simulink model "ElectricVehicleThermalManagementWithHeatPump"  (R2024b)
settings: Solver=VariableStepAuto  StartTime=0.0  StopTime=3600  RelTol=1e-3  AbsTol=1e-3
PreLoadFcn:
  | init_nmpc
InitFcn:
  | init_nmpc
model workspace: external: MATLAB File ElectricVehicleThermalManagementWithHeatPumpParameters.m (data not in the file)
values from neighbouring files (symbols this model uses):
  battery_C1_LUT = [1913.6 12447 30609 ... (first row only)    [ElectricVehicleThermalManagementWithHeatPumpParameters.m]
  battery_capacity_LUT = [280.081 276.25 276.392]    [ElectricVehicleThermalManagementWithHeatPumpParameters.m]
  battery_cell_cp = 795    [ElectricVehicleThermalManagementWithHeatPumpParameters.m]
  battery_cell_mass = 2.5    [ElectricVehicleThermalManagementWithHeatPumpParameters.m]
  battery_Em_LUT = [3.4966 3.5057 3.5148 ... (first row only)    [ElectricVehicleThermalManagementWithHeatPumpParameters.m]
  battery_N_cells = 20    [ElectricVehicleThermalManagementWithHeatPumpParameters.m]
  battery_Qe_init = 0    [ElectricVehicleThermalManagementWithHeatPumpParameters.m]
  battery_R0_LUT = [0.0117 0.0085 0.009 ... (first row only)    [ElectricVehicleThermalManagementWithHeatPumpParameters.m]
  battery_R1_LUT = [0.0109 0.0029 0.0013 ... (first row only)    [ElectricVehicleThermalManagementWithHeatPumpParameters.m]
  battery_SOC_LUT = [0; 0.1; 0.25; 0.5; 0.75; 0.9; 1]    [ElectricVehicleThermalManagementWithHeatPumpParameters.m]
  battery_T_init = -10    [ElectricVehicleThermalManagementWithHeatPumpParameters.m]
  battery_temperature_LUT = [5 20 40]    [ElectricVehicleThermalManagementWithHeatPumpParameters.m]
  cabin_duct_area = 0.04    [ElectricVehicleThermalManagementWithHeatPumpParameters.m]
  cabin_T_init = -10    [ElectricVehicleThermalManagementWithHeatPumpParameters.m]
  chiller_area_primary = 0.43982297150257105    (= 0.439822971503)    [ElectricVehicleThermalManagementWithHeatPumpParameters.m]
  chiller_N_baffles = 3    [ElectricVehicleThermalManagementWithHeatPumpParameters.m]
  chiller_N_tubes = 100    [ElectricVehicleThermalManagementWithHeatPumpParameters.m]
  chiller_tube_D = 0.0035    [ElectricVehicleThermalManagementWithHeatPumpParameters.m]
  chiller_tube_L = 0.4    [ElectricVehicleThermalManagementWithHeatPumpParameters.m]
  chiller_wall_conductivity = 240    [ElectricVehicleThermalManagementWithHeatPumpParameters.m]
  chiller_wall_thickness = 0.0001    [ElectricVehicleThermalManagementWithHeatPumpParameters.m]
  cond_evap_air_area_flow = 0.3906    [ElectricVehicleThermalManagementWithHeatPumpParameters.m]
  cond_evap_air_area_primary = 1.4834999999999998    (= 1.4835)    [ElectricVehicleThermalManagementWithHeatPumpParameters.m]
  cond_evap_W = 0.015    [ElectricVehicleThermalManagementWithHeatPumpParameters.m]
  cond_evap_wall_conductivity = 240    [ElectricVehicleThermalManagementWithHeatPumpParameters.m]
  cond_evap_wall_thickness = 0.0001    [ElectricVehicleThermalManagementWithHeatPumpParameters.m]
  coolant_channel_D = 0.0092    [ElectricVehicleThermalManagementWithHeatPumpParameters.m]
  coolant_pipe_D = 0.019    [ElectricVehicleThermalManagementWithHeatPumpParameters.m]
  coolant_T_init = -10    [ElectricVehicleThermalManagementWithHeatPumpParameters.m]
  coolant_tank_area = 0.0121    [ElectricVehicleThermalManagementWithHeatPumpParameters.m]
  coolant_tank_volume = 1.25    [ElectricVehicleThermalManagementWithHeatPumpParameters.m]
  coolant_valve_D_ratio_max = 0.95    [ElectricVehicleThermalManagementWithHeatPumpParameters.m]
  coolant_valve_D_ratio_min = 0.001    [ElectricVehicleThermalManagementWithHeatPumpParameters.m]
  coolant_valve_displacement = 0.0063    [ElectricVehicleThermalManagementWithHeatPumpParameters.m]
  coolant_valve_S_max = 0.0053    [ElectricVehicleThermalManagementWithHeatPumpParameters.m]
  evaporator_air_area_flow = 0.12    [ElectricVehicleThermalManagementWithHeatPumpParameters.m]
  evaporator_air_area_primary = 0.4323    [ElectricVehicleThermalManagementWithHeatPumpParameters.m]
  evaporator_W = 0.015    [ElectricVehicleThermalManagementWithHeatPumpParameters.m]
  evaporator_wall_conductivity = 240    [ElectricVehicleThermalManagementWithHeatPumpParameters.m]
  evaporator_wall_thickness = 0.0001    [ElectricVehicleThermalManagementWithHeatPumpParameters.m]
  expansion_valve_D_ratio_max = 0.9    [ElectricVehicleThermalManagementWithHeatPumpParameters.m]
  hex_area_primary = 0.070371675440411369    (= 0.0703716754404)    [ElectricVehicleThermalManagementWithHeatPumpParameters.m]
  hex_N_tubes = 64    [ElectricVehicleThermalManagementWithHeatPumpParameters.m]
  hex_tube_D = 0.0035    [ElectricVehicleThermalManagementWithHeatPumpParameters.m]
  hex_wall_conductivity = 240    [ElectricVehicleThermalManagementWithHeatPumpParameters.m]
  hex_wall_thickness = 0.0001    [ElectricVehicleThermalManagementWithHeatPumpParameters.m]
  inner_cond_air_area_flow = 0.1953    [ElectricVehicleThermalManagementWithHeatPumpParameters.m]
  inner_cond_air_area_primary = 0.99520000000000008    (= 0.9952)    [ElectricVehicleThermalManagementWithHeatPumpParameters.m]
  inner_cond_W = 0.02    [ElectricVehicleThermalManagementWithHeatPumpParameters.m]
  inner_cond_wall_conductivity = 240    [ElectricVehicleThermalManagementWithHeatPumpParameters.m]
  inner_cond_wall_thickness = 0.0001    [ElectricVehicleThermalManagementWithHeatPumpParameters.m]
  pump_speed_max = 1000    [ElectricVehicleThermalManagementWithHeatPumpParameters.m]
  radiator_air_area_flow = 0.097499999999999989    (= 0.0975)    [ElectricVehicleThermalManagementWithHeatPumpParameters.m]
  radiator_air_area_primary = 0.43687499999999996    (= 0.436875)    [ElectricVehicleThermalManagementWithHeatPumpParameters.m]
  radiator_W = 0.015    [ElectricVehicleThermalManagementWithHeatPumpParameters.m]
  radiator_wall_conductivity = 240    [ElectricVehicleThermalManagementWithHeatPumpParameters.m]
  radiator_wall_thickness = 0.0001    [ElectricVehicleThermalManagementWithHeatPumpParameters.m]
  refrigerant_p_init = 0.2    [ElectricVehicleThermalManagementWithHeatPumpParameters.m]
  refrigerant_pipe_D = 0.01    [ElectricVehicleThermalManagementWithHeatPumpParameters.m]
  refrigerant_valve_D_ratio_max = 0.95    [ElectricVehicleThermalManagementWithHeatPumpParameters.m]
  refrigerant_valve_displacement = 0.005    [ElectricVehicleThermalManagementWithHeatPumpParameters.m]
libraries: fl_lib x227, nesl_utility x162, SimscapeFluids_lib x30, LiBatteryElements_lib x16, slpidlib x3, SignalEditorBlockLib x1
(part 1 of 13)
CloseFcn:
  | try,close(h1_ElectricVehicleThermalManagementWithHeatPump),end
  | clear h1_ElectricVehicleThermalManagementWithHeatPump
  | 
  | clear tout simlog_ElectricVehicleThermalManagementWithHeatPump
  | clear tout simlog_ElectricVehicleThermalManagementWithHeatPump
Description:
  | Electric Vehicle Thermal Management With Heat Pump
settings Model: Creator=The MathWorks, Inc.  LastModifiedBy=prashant.lokur
settings SolverCC: AutoScaleAbsTol=off  MaxConsecutiveMinStep=2  AlgebraicLoopSolver=TrustRegion  MaxZcPerStep=1
settings DataIOCC: InspectSignalLogs=on
settings DebuggingCC: UnconnectedInputMsg=warning  UnconnectedOutputMsg=warning  UnconnectedLineMsg=warning  SymbolicDimsDataTypeCodeGenerationDiagnostic=none
settings ModelReferenceCC: EnableRefExpFcnMdlSchedulingChecks=on
settings SFSimCC: CustomCodeUndefinedFunction=UseInterfaceOnly
settings RTWCC: GPUComputeCapability=3.5  DLArmComputeVersion=19.05
settings SimscapeCC: EditingMode=Restricted  SimscapeLogType=all  SimscapeLogSimulationStatistics=on  SimscapeLogName=simlog_ElectricVehicleThermalManagementWithHeatPump  SimscapeLogLimitData=off  SimscapeLogDataHistory=20000

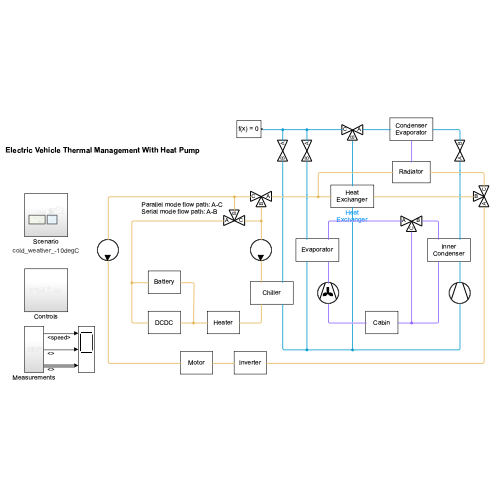
[thumbnail: Simulink's stored preview of the top-level diagram]
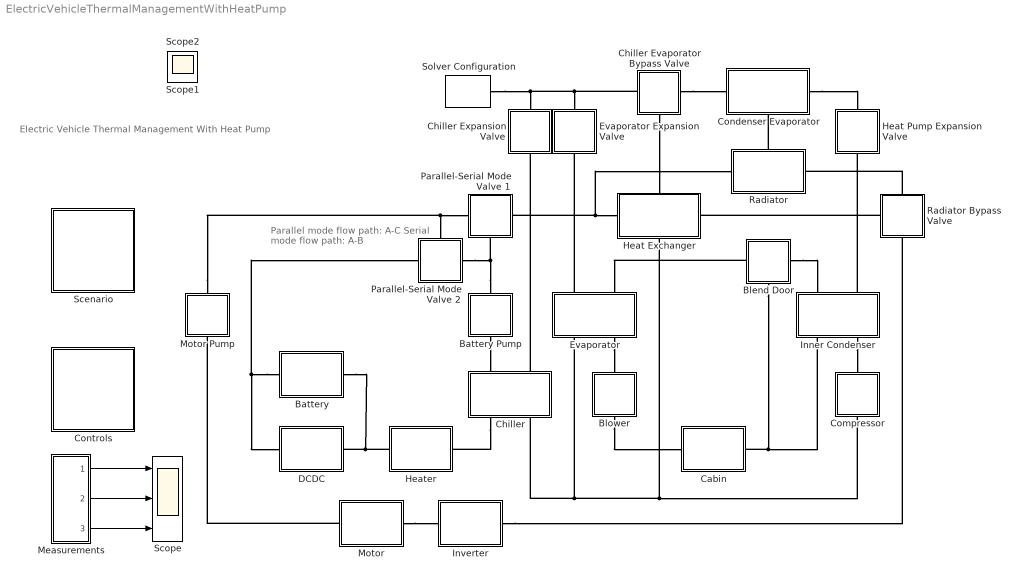
== system ElectricVehicleThermalManagementWithHeatPump ==
  note: Electric Vehicle Thermal Management With Heat Pump
  note: Parallel mode flow path: A-C
      | Serial mode flow path: A-B
  Battery : Subsystem  Tag=PublishSubsystem
      mask Display: disp(get_param(gcb, 'Name'))
  Battery Pump : Subsystem
      settings: PortSchema="{\"entries\":[{\"content\":{\"sides\":[{\"content\":{},\"type\":\"ConnectorPlacement.EquallySpacedRectSide\",\"uuid\":\"8608e54e-2c97-4e6c-91d5-e9fd83f4c634\"},{\"content\":{\"side\":\"RIGHT\"},\"type\":\"ConnectorPlacement.EquallySpacedRectSide\",\"uuid\":\"2094794e-7928-4a36-8d26-6d0877832239\"},{\"content\":{\"connectorIds\":[\"LConn1\"],\"side\":\"TOP\"},\"type\":\"ConnectorPlacement.EquallySpacedRectSide\",\"uuid\":\"5d2e6c3a-6919-4acd-9f23-628827b4d5b1\"},{\"content\":{\"connectorIds\":[\"RConn1\"],\"side\":\"BOTTOM\"},\"type\":\"ConnectorPlacement.EquallySpacedRectSide\",\"uuid\":\"7eb8f1d1-21e2-47d8-bcb5-892664c8f83c\"}]},\"type\":\"ConnectorPlacement.EquallySpacedConnector\",\"uuid\":\"45db803b-5189-4980-a07c-fba0b10a9ca2\"}],\"packageUris\":[\"http://schema.mathworks.com/mf0/Connector/R2020b\"],\"version\":\"1.0\"}"
      mask Display:
      | plot(100*cos(linspace(0, 2*pi, 500)), 100*sin(linspace(0, 2*pi, 500)))
      | patch([0 24 -24 0], [-100 -55 -55 -100]+1, [0 0 0])
  Blend Door : Subsystem
      settings: PortSchema="{\"entries\":[{\"content\":{\"sides\":[{\"content\":{\"connectorIds\":[\"LConn1\"]},\"type\":\"ConnectorPlacement.EquallySpacedRectSide\",\"uuid\":\"8608e54e-2c97-4e6c-91d5-e9fd83f4c634\"},{\"content\":{\"connectorIds\":[\"RConn1\"],\"side\":\"RIGHT\"},\"type\":\"ConnectorPlacement.EquallySpacedRectSide\",\"uuid\":\"2094794e-7928-4a36-8d26-6d0877832239\"},{\"content\":{\"side\":\"TOP\"},\"type\":\"ConnectorPlacement.EquallySpacedRectSide\",\"uuid\":\"5d2e6c3a-6919-4acd-9f23-628827b4d5b1\"},{\"content\":{\"connectorIds\":[\"RConn2\"],\"side\":\"BOTTOM\"},\"type\":\"ConnectorPlacement.EquallySpacedRectSide\",\"uuid\":\"12f1c895-2983-4276-b305-f1b4f2b8f289\"}]},\"type\":\"ConnectorPlacement.EquallySpacedConnector\",\"uuid\":\"45db803b-5189-4980-a07c-fba0b10a9ca2\"}],\"packageUris\":[\"http://schema.mathworks.com/mf0/Connector/R2020b\"],\"version\":\"1.0\"}"
      mask Display:
      | color('white')
      | plot(100, 100)
      | plot(-100, -100)
      | color('black')
      | 
      | plot([0 -100 -100 0], [0 50 -50 0])
      | plot([0 100 100 0], [0 50 -50 0])
      | plot([0 50 -50 0], [0 -100 -100 0])
  Blower : Subsystem  Tag=PublishSubsystem
      settings: PortSchema="{\"entries\":[{\"content\":{\"sides\":[{\"content\":{},\"type\":\"ConnectorPlacement.EquallySpacedRectSide\",\"uuid\":\"8608e54e-2c97-4e6c-91d5-e9fd83f4c634\"},{\"content\":{\"side\":\"RIGHT\"},\"type\":\"ConnectorPlacement.EquallySpacedRectSide\",\"uuid\":\"2094794e-7928-4a36-8d26-6d0877832239\"},{\"content\":{\"connectorIds\":[\"LConn1\"],\"side\":\"TOP\"},\"type\":\"ConnectorPlacement.EquallySpacedRectSide\",\"uuid\":\"5d2e6c3a-6919-4acd-9f23-628827b4d5b1\"},{\"content\":{\"connectorIds\":[\"RConn1\"],\"side\":\"BOTTOM\"},\"type\":\"ConnectorPlacement.EquallySpacedRectSide\",\"uuid\":\"c4235038-bb07-402c-a25d-479cdb2413d7\"}]},\"type\":\"ConnectorPlacement.EquallySpacedConnector\",\"uuid\":\"45db803b-5189-4980-a07c-fba0b10a9ca2\"}],\"packageUris\":[\"http://schema.mathworks.com/mf0/Connector/R2020b\"],\"version\":\"1.0\"}"
      mask Display:
      | plot(100*cos(linspace(0, 2*pi, 500)), 100*sin(linspace(0, 2*pi, 500)))
      | plot([28 80], [96 -60])
      | plot([-28 -80], [96 -60])
      | patch(-50*sin(3*linspace(0, pi, 500)).*cos(linspace(0, pi, 500)), -50*sin(3*linspace(0, pi, 500)).*sin(linspace(0, pi, 500)), [0 0 0])
  Cabin : Subsystem  Tag=PublishSubsystem
      mask Display: disp(get_param(gcb, 'Name'))
  Chiller : Subsystem  Tag=PublishSubsystem
      settings: PortSchema="{\"entries\":[{\"content\":{\"sides\":[{\"content\":{},\"type\":\"ConnectorPlacement.EquallySpacedRectSide\",\"uuid\":\"08dd7f1a-2c57-4e0b-bc0c-3dc595a62f47\"},{\"content\":{\"side\":\"RIGHT\"},\"type\":\"ConnectorPlacement.EquallySpacedRectSide\",\"uuid\":\"ff3adbe6-50e6-4ee9-89c8-33b172e39e14\"},{\"content\":{\"connectorIds\":[\"LConn1\",\"LConn2\"],\"side\":\"TOP\"},\"type\":\"ConnectorPlacement.EquallySpacedRectSide\",\"uuid\":\"dbd0f117-c61e-4d8b-a34c-15c789eeb10d\"},{\"content\":{\"connectorIds\":[\"RConn1\",\"RConn2\"],\"side\":\"BOTTOM\"},\"type\":\"ConnectorPlacement.EquallySpacedRectSide\",\"uuid\":\"0d4c84fc-b13c-4ee0-9956-2ee11d67b2ad\"}]},\"type\":\"ConnectorPlacement.EquallySpacedConnector\",\"uuid\":\"74c2ffb8-8fce-48fb-ac7c-d547444760e2\"}],\"packageUris\":[\"http://schema.mathworks.com/mf0/Connector/R2020b\"],\"version\":\"1.0\"}"
      mask Display: disp(get_param(gcb, 'Name'))
  Chiller Expansion Valve : Subsystem  Tag=PublishSubsystem
      settings: PortSchema="{\"entries\":[{\"content\":{\"sides\":[{\"content\":{},\"type\":\"ConnectorPlacement.EquallySpacedRectSide\",\"uuid\":\"8608e54e-2c97-4e6c-91d5-e9fd83f4c634\"},{\"content\":{\"side\":\"RIGHT\"},\"type\":\"ConnectorPlacement.EquallySpacedRectSide\",\"uuid\":\"2094794e-7928-4a36-8d26-6d0877832239\"},{\"content\":{\"connectorIds\":[\"LConn1\"],\"side\":\"TOP\"},\"type\":\"ConnectorPlacement.EquallySpacedRectSide\",\"uuid\":\"5d2e6c3a-6919-4acd-9f23-628827b4d5b1\"},{\"content\":{\"connectorIds\":[\"RConn1\"],\"side\":\"BOTTOM\"},\"type\":\"ConnectorPlacement.EquallySpacedRectSide\",\"uuid\":\"5466525f-0f04-4dbe-888f-4c3dddfbc528\"}]},\"type\":\"ConnectorPlacement.EquallySpacedConnector\",\"uuid\":\"45db803b-5189-4980-a07c-fba0b10a9ca2\"}],\"packageUris\":[\"http://schema.mathworks.com/mf0/Connector/R2020b\"],\"version\":\"1.0\"}"
      mask Display:
      | color('white')
      | plot(100, 100)
      | plot(-100, -100)
      | color('black')
      | 
      | plot([0 50 -50 0], [0 -100 -100 0])
      | plot([0 50 -50 0], [0 100 100 0])
  Chiller Evaporator Bypass Valve : Subsystem  Tag=PublishSubsystem
      settings: PortSchema="{\"entries\":[{\"content\":{\"sides\":[{\"content\":{\"connectorIds\":[\"LConn1\"]},\"type\":\"ConnectorPlacement.EquallySpacedRectSide\",\"uuid\":\"8608e54e-2c97-4e6c-91d5-e9fd83f4c634\"},{\"content\":{\"connectorIds\":[\"RConn1\"],\"side\":\"RIGHT\"},\"type\":\"ConnectorPlacement.EquallySpacedRectSide\",\"uuid\":\"2094794e-7928-4a36-8d26-6d0877832239\"},{\"content\":{\"side\":\"TOP\"},\"type\":\"ConnectorPlacement.EquallySpacedRectSide\",\"uuid\":\"5d2e6c3a-6919-4acd-9f23-628827b4d5b1\"},{\"content\":{\"connectorIds\":[\"RConn2\"],\"side\":\"BOTTOM\"},\"type\":\"ConnectorPlacement.EquallySpacedRectSide\",\"uuid\":\"12f1c895-2983-4276-b305-f1b4f2b8f289\"}]},\"type\":\"ConnectorPlacement.EquallySpacedConnector\",\"uuid\":\"45db803b-5189-4980-a07c-fba0b10a9ca2\"}],\"packageUris\":[\"http://schema.mathworks.com/mf0/Connector/R2020b\"],\"version\":\"1.0\"}"
      mask Display:
      | color('white')
      | plot(100, 100)
      | plot(-100, -100)
      | color('black')
      | 
      | plot([0 -100 -100 0], [0 50 -50 0])
      | plot([0 100 100 0], [0 50 -50 0])
      | plot([0 50 -50 0], [0 -100 -100 0])
  Compressor : Subsystem  Tag=PublishSubsystem
      settings: PortSchema="{\"entries\":[{\"content\":{\"sides\":[{\"content\":{},\"type\":\"ConnectorPlacement.EquallySpacedRectSide\",\"uuid\":\"8608e54e-2c97-4e6c-91d5-e9fd83f4c634\"},{\"content\":{\"side\":\"RIGHT\"},\"type\":\"ConnectorPlacement.EquallySpacedRectSide\",\"uuid\":\"2094794e-7928-4a36-8d26-6d0877832239\"},{\"content\":{\"connectorIds\":[\"LConn1\"],\"side\":\"TOP\"},\"type\":\"ConnectorPlacement.EquallySpacedRectSide\",\"uuid\":\"5d2e6c3a-6919-4acd-9f23-628827b4d5b1\"},{\"content\":{\"connectorIds\":[\"RConn1\"],\"side\":\"BOTTOM\"},\"type\":\"ConnectorPlacement.EquallySpacedRectSide\",\"uuid\":\"ed0a8ac6-4625-4be3-8c8e-84380e16051c\"}]},\"type\":\"ConnectorPlacement.EquallySpacedConnector\",\"uuid\":\"45db803b-5189-4980-a07c-fba0b10a9ca2\"}],\"packageUris\":[\"http://schema.mathworks.com/mf0/Connector/R2020b\"],\"version\":\"1.0\"}"
      mask Display:
      | plot(100*cos(linspace(0, 2*pi, 500)), 100*sin(linspace(0, 2*pi, 500)))
      | plot([28 80], [96 -60])
      | plot([-28 -80], [96 -60])
  Condenser Evaporator : Subsystem  Tag=PublishSubsystem
      settings: PortSchema="{\"entries\":[{\"content\":{\"sides\":[{\"content\":{\"connectorIds\":[\"LConn1\"]},\"type\":\"ConnectorPlacement.EquallySpacedRectSide\",\"uuid\":\"07c3df60-ca73-4a82-8a74-bbe62fbe14d4\"},{\"content\":{\"connectorIds\":[\"RConn1\"],\"side\":\"RIGHT\"},\"type\":\"ConnectorPlacement.EquallySpacedRectSide\",\"uuid\":\"9db9ae49-9d94-4ce4-9f2f-75754f4c26b5\"},{\"content\":{\"side\":\"TOP\"},\"type\":\"ConnectorPlacement.EquallySpacedRectSide\",\"uuid\":\"fd8c0c23-133d-46ca-bac8-f53d714a10c9\"},{\"content\":{\"connectorIds\":[\"RConn2\"],\"side\":\"BOTTOM\"},\"type\":\"ConnectorPlacement.EquallySpacedRectSide\",\"uuid\":\"1982af02-f04e-4e44-9cd8-4410768eed4d\"}]},\"type\":\"ConnectorPlacement.EquallySpacedConnector\",\"uuid\":\"8e0ae7db-f1f8-46e5-b300-69983ccb91b0\"}],\"packageUris\":[\"http://schema.mathworks.com/mf0/Connector/R2020b\"],\"version\":\"1.0\"}"
      mask Display: disp(get_param(gcb, 'Name'))
  Controls : Subsystem  Tag=PublishSubsystem
  DCDC : Subsystem
      mask Display: disp(get_param(gcb, 'Name'))
  Evaporator : Subsystem  Tag=PublishSubsystem
      settings: PortSchema="{\"entries\":[{\"content\":{\"sides\":[{\"content\":{},\"type\":\"ConnectorPlacement.EquallySpacedRectSide\",\"uuid\":\"08dd7f1a-2c57-4e0b-bc0c-3dc595a62f47\"},{\"content\":{\"side\":\"RIGHT\"},\"type\":\"ConnectorPlacement.EquallySpacedRectSide\",\"uuid\":\"ff3adbe6-50e6-4ee9-89c8-33b172e39e14\"},{\"content\":{\"connectorIds\":[\"LConn1\",\"LConn2\"],\"side\":\"TOP\"},\"type\":\"ConnectorPlacement.EquallySpacedRectSide\",\"uuid\":\"dbd0f117-c61e-4d8b-a34c-15c789eeb10d\"},{\"content\":{\"connectorIds\":[\"RConn1\",\"RConn2\"],\"side\":\"BOTTOM\"},\"type\":\"ConnectorPlacement.EquallySpacedRectSide\",\"uuid\":\"a1739911-191b-44a6-b898-cc4889767178\"}]},\"type\":\"ConnectorPlacement.EquallySpacedConnector\",\"uuid\":\"74c2ffb8-8fce-48fb-ac7c-d547444760e2\"}],\"packageUris\":[\"http://schema.mathworks.com/mf0/Connector/R2020b\"],\"version\":\"1.0\"}"
      mask Display: disp(get_param(gcb, 'Name'))
  Evaporator Expansion Valve : Subsystem  Tag=PublishSubsystem
      settings: PortSchema="{\"entries\":[{\"content\":{\"sides\":[{\"content\":{},\"type\":\"ConnectorPlacement.EquallySpacedRectSide\",\"uuid\":\"8608e54e-2c97-4e6c-91d5-e9fd83f4c634\"},{\"content\":{\"side\":\"RIGHT\"},\"type\":\"ConnectorPlacement.EquallySpacedRectSide\",\"uuid\":\"2094794e-7928-4a36-8d26-6d0877832239\"},{\"content\":{\"connectorIds\":[\"LConn1\"],\"side\":\"TOP\"},\"type\":\"ConnectorPlacement.EquallySpacedRectSide\",\"uuid\":\"5d2e6c3a-6919-4acd-9f23-628827b4d5b1\"},{\"content\":{\"connectorIds\":[\"RConn1\"],\"side\":\"BOTTOM\"},\"type\":\"ConnectorPlacement.EquallySpacedRectSide\",\"uuid\":\"dee56540-0438-4e4d-b3ab-37064a293584\"}]},\"type\":\"ConnectorPlacement.EquallySpacedConnector\",\"uuid\":\"45db803b-5189-4980-a07c-fba0b10a9ca2\"}],\"packageUris\":[\"http://schema.mathworks.com/mf0/Connector/R2020b\"],\"version\":\"1.0\"}"
      mask Display:
      | color('white')
      | plot(100, 100)
      | plot(-100, -100)
      | color('black')
      | 
      | plot([0 50 -50 0], [0 -100 -100 0])
      | plot([0 50 -50 0], [0 100 100 0])
  Heat Exchanger : Subsystem  Tag=PublishSubsystem
      settings: PortSchema="{\"entries\":[{\"content\":{\"sides\":[{\"content\":{\"connectorIds\":[\"LConn1\"]},\"type\":\"ConnectorPlacement.EquallySpacedRectSide\",\"uuid\":\"08dd7f1a-2c57-4e0b-bc0c-3dc595a62f47\"},{\"content\":{\"connectorIds\":[\"RConn1\"],\"side\":\"RIGHT\"},\"type\":\"ConnectorPlacement.EquallySpacedRectSide\",\"uuid\":\"ff3adbe6-50e6-4ee9-89c8-33b172e39e14\"},{\"content\":{\"connectorIds\":[\"LConn2\"],\"side\":\"TOP\"},\"type\":\"ConnectorPlacement.EquallySpacedRectSide\",\"uuid\":\"dbd0f117-c61e-4d8b-a34c-15c789eeb10d\"},{\"content\":{\"connectorIds\":[\"RConn2\"],\"side\":\"BOTTOM\"},\"type\":\"ConnectorPlacement.EquallySpacedRectSide\",\"uuid\":\"042be640-9063-45a3-8f14-0e35b2f9701a\"}]},\"type\":\"ConnectorPlacement.EquallySpacedConnector\",\"uuid\":\"74c2ffb8-8fce-48fb-ac7c-d547444760e2\"}],\"packageUris\":[\"http://schema.mathworks.com/mf0/Connector/R2020b\"],\"version\":\"1.0\"}"
      mask Display: disp(get_param(gcb, 'Name'))
  Heat Pump Expansion Valve : Subsystem  Tag=PublishSubsystem
      settings: PortSchema="{\"entries\":[{\"content\":{\"sides\":[{\"content\":{},\"type\":\"ConnectorPlacement.EquallySpacedRectSide\",\"uuid\":\"8608e54e-2c97-4e6c-91d5-e9fd83f4c634\"},{\"content\":{\"side\":\"RIGHT\"},\"type\":\"ConnectorPlacement.EquallySpacedRectSide\",\"uuid\":\"2094794e-7928-4a36-8d26-6d0877832239\"},{\"content\":{\"connectorIds\":[\"LConn1\"],\"side\":\"TOP\"},\"type\":\"ConnectorPlacement.EquallySpacedRectSide\",\"uuid\":\"5d2e6c3a-6919-4acd-9f23-628827b4d5b1\"},{\"content\":{\"connectorIds\":[\"RConn1\"],\"side\":\"BOTTOM\"},\"type\":\"ConnectorPlacement.EquallySpacedRectSide\",\"uuid\":\"a6d8b143-f5c4-47d8-b413-b9e61d8ce1dd\"}]},\"type\":\"ConnectorPlacement.EquallySpacedConnector\",\"uuid\":\"45db803b-5189-4980-a07c-fba0b10a9ca2\"}],\"packageUris\":[\"http://schema.mathworks.com/mf0/Connector/R2020b\"],\"version\":\"1.0\"}"
      mask Display:
      | color('white')
      | plot(100, 100)
      | plot(-100, -100)
      | color('black')
      | 
      | plot([0 50 -50 0], [0 -100 -100 0])
      | plot([0 50 -50 0], [0 100 100 0])
  Heater : Subsystem  Tag=PublishSubsystem
      mask Display: disp(get_param(gcb, 'Name'))
  Inner Condenser : Subsystem  Tag=PublishSubsystem
      settings: PortSchema="{\"entries\":[{\"content\":{\"sides\":[{\"content\":{},\"type\":\"ConnectorPlacement.EquallySpacedRectSide\",\"uuid\":\"08dd7f1a-2c57-4e0b-bc0c-3dc595a62f47\"},{\"content\":{\"side\":\"RIGHT\"},\"type\":\"ConnectorPlacement.EquallySpacedRectSide\",\"uuid\":\"ff3adbe6-50e6-4ee9-89c8-33b172e39e14\"},{\"content\":{\"connectorIds\":[\"LConn1\",\"LConn2\"],\"side\":\"TOP\"},\"type\":\"ConnectorPlacement.EquallySpacedRectSide\",\"uuid\":\"dbd0f117-c61e-4d8b-a34c-15c789eeb10d\"},{\"content\":{\"connectorIds\":[\"RConn1\",\"RConn2\"],\"side\":\"BOTTOM\"},\"type\":\"ConnectorPlacement.EquallySpacedRectSide\",\"uuid\":\"996ebcad-2560-47a7-9c56-3ae78dd46971\"}]},\"type\":\"ConnectorPlacement.EquallySpacedConnector\",\"uuid\":\"74c2ffb8-8fce-48fb-ac7c-d547444760e2\"}],\"packageUris\":[\"http://schema.mathworks.com/mf0/Connector/R2020b\"],\"version\":\"1.0\"}"
      mask Display: disp(get_param(gcb, 'Name'))
  Inverter : Subsystem
      mask Display: disp(get_param(gcb, 'Name'))
  Measurements : Subsystem
  Motor : Subsystem  Tag=PublishSubsystem
      mask Display: disp(get_param(gcb, 'Name'))
  Motor Pump : Subsystem  Tag=PublishSubsystem
      settings: PortSchema="{\"entries\":[{\"content\":{\"sides\":[{\"content\":{},\"type\":\"ConnectorPlacement.EquallySpacedRectSide\",\"uuid\":\"8608e54e-2c97-4e6c-91d5-e9fd83f4c634\"},{\"content\":{\"side\":\"RIGHT\"},\"type\":\"ConnectorPlacement.EquallySpacedRectSide\",\"uuid\":\"2094794e-7928-4a36-8d26-6d0877832239\"},{\"content\":{\"connectorIds\":[\"LConn1\"],\"side\":\"TOP\"},\"type\":\"ConnectorPlacement.EquallySpacedRectSide\",\"uuid\":\"5d2e6c3a-6919-4acd-9f23-628827b4d5b1\"},{\"content\":{\"connectorIds\":[\"RConn1\"],\"side\":\"BOTTOM\"},\"type\":\"ConnectorPlacement.EquallySpacedRectSide\",\"uuid\":\"33b18e2e-1f33-4985-aa8c-29c4f8ccc63e\"}]},\"type\":\"ConnectorPlacement.EquallySpacedConnector\",\"uuid\":\"45db803b-5189-4980-a07c-fba0b10a9ca2\"}],\"packageUris\":[\"http://schema.mathworks.com/mf0/Connector/R2020b\"],\"version\":\"1.0\"}"
      mask Display:
      | plot(100*cos(linspace(0, 2*pi, 500)), 100*sin(linspace(0, 2*pi, 500)))
      | patch([0 24 -24 0], [-100 -55 -55 -100]+1, [0 0 0])
  Parallel-Serial Mode Valve 1 : Subsystem  Tag=PublishSubsystem
      settings: PortSchema="{\"entries\":[{\"content\":{\"sides\":[{\"content\":{\"connectorIds\":[\"LConn1\"]},\"type\":\"ConnectorPlacement.EquallySpacedRectSide\",\"uuid\":\"701091b4-901c-43e1-a8a1-50bf4fd327d1\"},{\"content\":{\"connectorIds\":[\"RConn1\"],\"side\":\"RIGHT\"},\"type\":\"ConnectorPlacement.EquallySpacedRectSide\",\"uuid\":\"6ee33cdd-bbd1-4683-8a8c-22edb39550e2\"},{\"content\":{\"side\":\"TOP\"},\"type\":\"ConnectorPlacement.EquallySpacedRectSide\",\"uuid\":\"c0b8be11-b43c-4098-95a0-d44066221ea6\"},{\"content\":{\"connectorIds\":[\"RConn2\"],\"side\":\"BOTTOM\"},\"type\":\"ConnectorPlacement.EquallySpacedRectSide\",\"uuid\":\"08745159-a473-4b1a-b64e-559ffda253bb\"}]},\"type\":\"ConnectorPlacement.EquallySpacedConnector\",\"uuid\":\"9280612b-569a-4615-9ade-e87314c5223e\"}],\"packageUris\":[\"http://schema.mathworks.com/mf0/Connector/R2020b\"],\"version\":\"1.0\"}"
      mask Display:
      | color('white')
      | plot(100, 100)
      | plot(-100, -100)
      | color('black')
      | 
      | plot([0 -100 -100 0], [0 50 -50 0])
      | plot([0 100 100 0], [0 50 -50 0])
      | plot([0 50 -50 0], [0 -100 -100 0])
  Parallel-Serial Mode Valve 2 : Subsystem
      settings: PortSchema="{\"entries\":[{\"content\":{\"sides\":[{\"content\":{\"connectorIds\":[\"LConn1\"]},\"type\":\"ConnectorPlacement.EquallySpacedRectSide\",\"uuid\":\"07c3df60-ca73-4a82-8a74-bbe62fbe14d4\"},{\"content\":{\"connectorIds\":[\"RConn1\"],\"side\":\"RIGHT\"},\"type\":\"ConnectorPlacement.EquallySpacedRectSide\",\"uuid\":\"9db9ae49-9d94-4ce4-9f2f-75754f4c26b5\"},{\"content\":{\"connectorIds\":[\"LConn2\"],\"side\":\"TOP\"},\"type\":\"ConnectorPlacement.EquallySpacedRectSide\",\"uuid\":\"fd8c0c23-133d-46ca-bac8-f53d714a10c9\"}]},\"type\":\"ConnectorPlacement.EquallySpacedConnector\",\"uuid\":\"8e0ae7db-f1f8-46e5-b300-69983ccb91b0\"}],\"packageUris\":[\"http://schema.mathworks.com/mf0/Connector/R2020b\"],\"version\":\"1.0\"}"
      mask Display:
      | color('white')
      | plot(100, 100)
      | plot(-100, -100)
      | color('black')
      | 
      | plot([0 -100 -100 0], [0 50 -50 0])
      | plot([0 100 100 0], [0 50 -50 0])
      | plot([0 50 -50 0], [0 100 100 0])
  Radiator : Subsystem  Tag=PublishSubsystem
      settings: PortSchema="{\"entries\":[{\"content\":{\"sides\":[{\"content\":{\"connectorIds\":[\"LConn1\"]},\"type\":\"ConnectorPlacement.EquallySpacedRectSide\",\"uuid\":\"1c8aa983-a374-4f1b-b303-31d972477bc1\"},{\"content\":{\"connectorIds\":[\"RConn1\"],\"side\":\"RIGHT\"},\"type\":\"ConnectorPlacement.EquallySpacedRectSide\",\"uuid\":\"9470a7c4-8d01-4f33-b281-130c1633b9af\"},{\"content\":{\"connectorIds\":[\"LConn2\"],\"side\":\"TOP\"},\"type\":\"ConnectorPlacement.EquallySpacedRectSide\",\"uuid\":\"521bcd61-502e-4408-add3-862bd83fd72a\"},{\"content\":{\"connectorIds\":[],\"side\":\"HIDDEN\"},\"type\":\"ConnectorPlacement.EquallySpacedRectSide\",\"uuid\":\"1fd51896-89cd-4b86-8982-5d9c8888072c\"}]},\"type\":\"ConnectorPlacement.EquallySpacedConnector\",\"uuid\":\"d9db812f-15c4-4875-aa5b-4de8fb002b03\"}],\"packageUris\":[\"http://schema.mathworks.com/mf0/Connector/R2020b\"],\"version\":\"1.0\"}"
      mask Display: disp(get_param(gcb, 'Name'))
  Radiator Bypass Valve : Subsystem  Tag=PublishSubsystem
      settings: PortSchema="{\"entries\":[{\"content\":{\"sides\":[{\"content\":{\"connectorIds\":[\"LConn1\"]},\"type\":\"ConnectorPlacement.EquallySpacedRectSide\",\"uuid\":\"701091b4-901c-43e1-a8a1-50bf4fd327d1\"},{\"content\":{\"side\":\"RIGHT\"},\"type\":\"ConnectorPlacement.EquallySpacedRectSide\",\"uuid\":\"6ee33cdd-bbd1-4683-8a8c-22edb39550e2\"},{\"content\":{\"connectorIds\":[\"LConn2\"],\"side\":\"TOP\"},\"type\":\"ConnectorPlacement.EquallySpacedRectSide\",\"uuid\":\"c0b8be11-b43c-4098-95a0-d44066221ea6\"},{\"content\":{\"connectorIds\":[\"RConn1\"],\"side\":\"BOTTOM\"},\"type\":\"ConnectorPlacement.EquallySpacedRectSide\",\"uuid\":\"83027471-d1d2-4b40-ac40-09f8b2d5e483\"}]},\"type\":\"ConnectorPlacement.EquallySpacedConnector\",\"uuid\":\"9280612b-569a-4615-9ade-e87314c5223e\"}],\"packageUris\":[\"http://schema.mathworks.com/mf0/Connector/R2020b\"],\"version\":\"1.0\"}"
      mask Display:
      | color('white')
      | plot(100, 100)
      | plot(-100, -100)
      | color('black')
      | 
      | plot([0 -100 -100 0], [0 50 -50 0])
      | plot([0 50 -50 0], [0 100 100 0])
      | plot([0 50 -50 0], [0 -100 -100 0])
  Scenario : Subsystem  Tag=cold_weather_-10degC
      settings: AttributesFormatString=%<Tag>
  Scope : Scope  NumInputPorts=3
  Solver Configuration : nesl_utility/Solver Configuration  PhysicalDomain=network_engine_domain  SubClassName=solver  LeftPortType=input  RightPortType=generic  Tones=[]  Harmonics=[]  SimulateNoise=off  Profile=off  UseLocalSampling=off  EnableSwitchedLinearOptims=on  FrequencyDomain=off  UseCCode=off  RelTol=0.001  AbsTol=0.001  MinStep=1e-09  ToWorkspace=off  RevertToSquareIcSolve=off  NumHomotopyIterations=100  PhasorMode=off  PhasorModeNumHarmonics=1  ConsistencySolver=NEWTON_XTOL_AFTER_FTOL  IndexReductionMethod=DerivativeReplacement  DoDC=off  ResidualTolerance=1e-09  ConsistencyTolSource=GLOBAL  ConsistencyAbsTol=0.001  ConsistencyRelTol=0.001  ConsistencyTolFactor=0.001  UseLocalSolver=off  LocalSolverChoice=NE_BACKWARD_EULER_ADVANCER  ResolveIndetEquations=on  FunctionEvalNumThread=1  LocalSolverSampleTime=0.001  DoFixedCost=off  MaxNonlinIter=3  MaxModeIter=2  ComputeImpulses=off  ImpulseIterations=2  LinearAlgebra=auto  LinearAlgebraNumThread=0  EquationFormulation=NE_TIME_EF  DelaysMemoryBudget=1024  AutomaticFiltering=on  FilteringTimeConstant=0.001  PartitionStorageMethod=AS_NEEDED  PartitionMemoryBudget=1024  PartitionMethod=ROBUST  MultibodyUseLocalSolver=off  MultibodyLocalSolverChoice=ODE1  MultibodyLocalSolverSampleTime=0.001
  Scope1 : Scope
  Scope2 : Scope
  wires:
  Measurements/1(Out1) -> Scope/1
  Measurements/2(Out2) -> Scope/2
  Measurements/3(Out5) -> Scope/3
  connections:
  Motor/RConn1 -- Inverter/LConn1
  Evaporator/RConn2 -- Blower/LConn1
  Blend Door/RConn2 -- Cabin/RConn1 -- Inner Condenser/RConn1
  Compressor/RConn1 -- Heat Exchanger/RConn2 -- Evaporator/RConn1 -- Chiller/RConn2
  Condenser Evaporator/RConn1 -- Heat Pump Expansion Valve/LConn1
  Evaporator/LConn1 -- Evaporator Expansion Valve/RConn1
  Inverter/RConn1 -- Radiator Bypass Valve/RConn1
  Parallel-Serial Mode Valve 1/RConn1 -- Heat Exchanger/LConn1 -- Radiator/LConn1
  Chiller/RConn1 -- Heater/RConn1
  Blower/RConn1 -- Cabin/LConn1
  Inner Condenser/RConn2 -- Compressor/LConn1
  Motor/LConn1 -- Motor Pump/RConn1
  Battery Pump/RConn1 -- Chiller/LConn1
  Blend Door/LConn1 -- Evaporator/LConn2
  Blend Door/RConn1 -- Inner Condenser/LConn1
  Chiller Evaporator Bypass Valve/RConn2 -- Heat Exchanger/LConn2
  Chiller Evaporator Bypass Valve/RConn1 -- Condenser Evaporator/LConn1
  Radiator Bypass Valve/LConn1 -- Heat Exchanger/RConn1
  Radiator Bypass Valve/LConn2 -- Radiator/RConn1
  Motor Pump/LConn1 -- Parallel-Serial Mode Valve 2/LConn2 -- Parallel-Serial Mode Valve 1/LConn1
  Battery Pump/LConn1 -- Parallel-Serial Mode Valve 2/RConn1 -- Parallel-Serial Mode Valve 1/RConn2
  Chiller Evaporator Bypass Valve/LConn1 -- Evaporator Expansion Valve/LConn1 -- Chiller Expansion Valve/LConn1 -- Solver Configuration/RConn1
  Chiller/LConn2 -- Chiller Expansion Valve/RConn1
  Inner Condenser/LConn2 -- Heat Pump Expansion Valve/RConn1
  Radiator/LConn2 -- Condenser Evaporator/RConn2
  Battery/LConn1 -- Parallel-Serial Mode Valve 2/LConn1 -- DCDC/LConn1
  Heater/LConn1 -- Battery/RConn1 -- DCDC/RConn1

== system ElectricVehicleThermalManagementWithHeatPump/Battery ==
  Coolant Jacket {1..4} (4 alike) : SimscapeFluids_lib/Thermal Liquid/Pipes & Fittings/Pipe (TL)  dynamic_compressibility=simscape.enum.onoff.on  inertia=simscape.enum.onoff.off  num_segments=1  pipe_length=0.7 m  cross_section_geometry=fluids.thermal_liquid.pipes_fittings.enum.CrossSectionGeometry.Custom  pipe_diameter=0.1 m  pipe_inner_diameter=0.05 m  pipe_outer_diameter=0.1 m  pipe_width=0.1 m  pipe_height=0.1 m  pipe_major_axis=0.1 m  pipe_minor_axis=0.05 m  pipe_side=0.1 m  pipe_angle=30 deg  area=pi * coolant_channel_D^2 / 4 m^2  Dh=coolant_channel_D m  elevation_spec=foundation.enum.constant_variable.constant  elevation_gain=0 m  gravity_spec=foundation.enum.constant_variable.constant  g=9.81 m/s^2  pressure_loss_spec=fluids.thermal_liquid.pipes_fittings.enum.PressureLossSpec.Haaland  local_pressure_loss_spec=fluids.thermal_liquid.pipes_fittings.enum.LocalLossSpec.AggregateLength  length_add=0 m  loss_coefficient=0.1  roughness_spec=fluids.thermal_liquid.pipes_fittings.enum.RoughnessSpec.Custom  roughness=1.5e-5 m  Re_friction_TLU=[ 400 1000 1.5e+3 3e+3 4e+3 6e+3 1e+4 2e+4 4e+4 6e+4 1e+5 1e+8 ]  friction_factor_TLU=[ 0.264 0.112 0.07099999999999999 0.0417 0.0387 0.0268 0.025 0.0232 0.0226 0.022 0.0214 0.0214 ]  Re_lam=100  Re_tur=500  shape_factor=64  mdot_nominal=[ 0.1 1 ] kg/s  p_diff_nominal=[ 0.001 0.01 ] MPa  mdot_threshold=1e-6 kg/s  wall_spec=fluids.thermal_liquid.pipes_fittings.enum.wall_spec.rigid  vol_expansion_spec=fluids.thermal_liquid.pipes_fittings.enum.VolumeExpansionSpec.Diameter  area_pressure_gain=1e-6 m^2/MPa  static_pressure_TLU=[.1, 1] MPa  area_pressure_gain_TLU=[1e-05, 1.1e-05] m^2  material_behavior_spec=fluids.thermal_liquid.pipes_fittings.enum.PipeMaterialBehavior.Linear  diameter_pressure_gain=1.2e-6 m/MPa  wall_thickness=0.05 m  elastic_modulus=69 GPa  stress_TLU=[276, 310] MPa  strain_TLU=[.004, .02]  stress_assert_action=simscape.enum.assert.action.none  stress_max=400 MPa  poisson_ratio=0.33  wall_time_constant=0.01 s  thermal_expansion=false  alpha_L_wall=24 um/(deltaK*m)  thermal_expansion_Tref=293.15 K  heat_transfer_spec=fluids.thermal_liquid.pipes_fittings.enum.HeatTransferSpec.DittusBoelter  mdot_nominal_heat=[ 0.1 1 ] kg/s  T_in_nominal=[ 293.15 293.15 ] K  T_out_nominal=[ 300 300 ] K  p_in_nominal_heat=[ 0.101325 0.101325 ] MPa  T_wall_nominal=[ 303.15 303.15 ] K  a_coeff=0.3  b_Re_power=0.8  c_Pr_power=0.33  Nu_lam=3.66  Re_Colburn_TLU=[ 100 150 1000 ]  Colburn_factor_TLU=[ 0.019 0.013 0.002 ]  Re_Nu_TLU=[ 100 150 1000 ]  Pr_Nu_TLU=[ 1 10 ]  Nu_TLU=[ 3.72 4.21; 3.75 4.44; 4.21 7.15 ]  p0_vec=coolant_p_init MPa  T0_vec=coolant_T_init degC  mdot0=0.1 kg/s
  Current Demand : fl_lib/Electrical/Electrical Sources/Controlled Current Source
  Electrical Reference : fl_lib/Electrical/Electrical Elements/Electrical Reference
  Flow Resistance (TL) : fl_lib/Thermal Liquid/Elements/Flow Resistance (TL)  delta_p_nominal=1e-5 MPa  mdot_nominal=0.02 kg/s  area=pi * coolant_pipe_D^2 / 4 m^2  laminar_fraction=1e-3
  Pack 1 : Subsystem  Tag=PublishSubsystem  mask(Lithium cell (one RC-branch equivalent circuit)){Ncells=30, Qe_init=battery_Qe_init, T_init=battery_T_init + 273.15, Capacity_LUT=battery_capacity_LUT, Em_LUT=battery_Em_LUT, R0_LUT=battery_R0_LUT, R1_LUT=battery_R1_LUT, C1_LUT=battery_C1_LUT, cell_mass=battery_cell_mass, cell_Cp_heat=battery_cell_cp, SOC_LUT=battery_SOC_LUT, Temperature_LUT=battery_temperature_LUT + 273.15}
      mask prompts: Ncells "Number of series-connected cells"; Qe_init "Initial cell charge deficit (A*hr)"; T_init "Initial cell temperature (K)"; Capacity_LUT "Capacity (A*hr, 1xN table)"; Em_LUT "Em open-circuit voltage, Em (volts, MxN table)"; R0_LUT "R0 terminal resistance (ohms, MxN table)"; R1_LUT "R1 cell resistance (ohms, MxN table)"; C1_LUT "C1 capacitance (farads, MxN table)"; cell_mass "Cell mass (kg)"; cell_Cp_heat "Cell specific heat (J/kg/K)"; SOC_LUT "SOC table breakpoints (Mx1 array)"; Temperature_LUT "Temperature table breakpoints (K, 1xN array)"
      mask DialogControl ParameterTabVar0 Prompt: Main
      mask DialogControl ParameterTabVar01 Prompt: Electrical (per cell)
      mask DialogControl ParameterTabVar012 Prompt: Thermal (per cell)
      mask DialogControl ParameterTabVar0123 Prompt: Table Breakpoints
      mask Display:
      | % Battery icon
      | plot([2.8 1.3], [0 0])
      | plot([-0.2 -1.2 -1.2 -2.8], [0 0 -0.8 -0.8])
      | patch([1 1 -1 -1]*0.15 + 1.6, [-1 1 1 -1]*0.4, [0 0 0])
      | patch([1 1 -1 -1]*0.15 + 0.4, [-1 1 1 -1]*0.4, [0 0 0])
      | patch([1 1 -1 -1]*0.15 + 1.0, [-1 1 1 -1]*0.8, [0 0 0])
      | patch([1 1 -1 -1]*0.15 - 0.2, [-1 1 1 -1]*0.8, [0 0 0])
      | 
      | % Thermal port
      | plot([-1.4 -0.8], [1.2 1.2])
      | plot([-1.4 -0.8], [0.5 0.5])
      | plot([-1.4 -2.8], [0.8 0.8])
      | plot(0.2*sin(0:2*pi/50:2*pi) - 1.4, 0.35*cos(0:2*pi/50:2*pi) + 0.85)
      | plot(0.2*sin(0:2*pi/50:pi) - 0.8, 0.35*cos(0:2*pi/50:pi) + 0.85)
      | 
      | % Plot points to set plot range
      | color('white')
      | plot(2.8, 1.6)
      | plot(-2.8, -1.6)
      | 
      | % Port labels
      | color('red')
      | port_label('LConn', 1, 'H')
      | port_label('LConn', 2, '+')
      | port_label('RConn', 1, '-')
  Pack 2 : Subsystem  mask(Lithium cell (one RC-branch equivalent circuit)){Ncells=battery_N_cells, Qe_init=battery_Qe_init, T_init=battery_T_init + 273.15, Capacity_LUT=battery_capacity_LUT, Em_LUT=battery_Em_LUT, R0_LUT=battery_R0_LUT, R1_LUT=battery_R1_LUT, C1_LUT=battery_C1_LUT, cell_mass=battery_cell_mass, cell_Cp_heat=battery_cell_cp, SOC_LUT=battery_SOC_LUT, Temperature_LUT=battery_temperature_LUT + 273.15}
      mask prompts: Ncells "Number of series-connected cells"; Qe_init "Initial cell charge deficit (A*hr)"; T_init "Initial cell temperature (K)"; Capacity_LUT "Capacity (A*hr, 1xN table)"; Em_LUT "Em open-circuit voltage, Em (volts, MxN table)"; R0_LUT "R0 terminal resistance (ohms, MxN table)"; R1_LUT "R1 cell resistance (ohms, MxN table)"; C1_LUT "C1 capacitance (farads, MxN table)"; cell_mass "Cell mass (kg)"; cell_Cp_heat "Cell specific heat (J/kg/K)"; SOC_LUT "SOC table breakpoints (Mx1 array)"; Temperature_LUT "Temperature table breakpoints (K, 1xN array)"
      mask DialogControl ParameterTabVar0 Prompt: Main
      mask DialogControl ParameterTabVar01 Prompt: Electrical (per cell)
      mask DialogControl ParameterTabVar012 Prompt: Thermal (per cell)
      mask DialogControl ParameterTabVar0123 Prompt: Table Breakpoints
      mask Display:
      | % Battery icon
      | plot([2.8 1.3], [0 0])
      | plot([-0.2 -1.2 -1.2 -2.8], [0 0 -0.8 -0.8])
      | patch([1 1 -1 -1]*0.15 + 1.6, [-1 1 1 -1]*0.4, [0 0 0])
      | patch([1 1 -1 -1]*0.15 + 0.4, [-1 1 1 -1]*0.4, [0 0 0])
      | patch([1 1 -1 -1]*0.15 + 1.0, [-1 1 1 -1]*0.8, [0 0 0])
      | patch([1 1 -1 -1]*0.15 - 0.2, [-1 1 1 -1]*0.8, [0 0 0])
      | 
      | % Thermal port
      | plot([-1.4 -0.8], [1.2 1.2])
      | plot([-1.4 -0.8], [0.5 0.5])
      | plot([-1.4 -2.8], [0.8 0.8])
      | plot(0.2*sin(0:2*pi/50:2*pi) - 1.4, 0.35*cos(0:2*pi/50:2*pi) + 0.85)
      | plot(0.2*sin(0:2*pi/50:pi) - 0.8, 0.35*cos(0:2*pi/50:pi) + 0.85)
      | 
      | % Plot points to set plot range
      | color('white')
      | plot(2.8, 1.6)
      | plot(-2.8, -1.6)
      | 
      | % Port labels
      | color('red')
      | port_label('LConn', 1, 'H')
      | port_label('LConn', 2, '+')
      | port_label('RConn', 1, '-')
  Pack 3 : Subsystem  mask(Lithium cell (one RC-branch equivalent circuit)){Ncells=battery_N_cells, Qe_init=battery_Qe_init, T_init=battery_T_init + 273.15, Capacity_LUT=battery_capacity_LUT, Em_LUT=battery_Em_LUT, R0_LUT=battery_R0_LUT, R1_LUT=battery_R1_LUT, C1_LUT=battery_C1_LUT, cell_mass=battery_cell_mass, cell_Cp_heat=battery_cell_cp, SOC_LUT=battery_SOC_LUT, Temperature_LUT=battery_temperature_LUT + 273.15}
      mask prompts: Ncells "Number of series-connected cells"; Qe_init "Initial cell charge deficit (A*hr)"; T_init "Initial cell temperature (K)"; Capacity_LUT "Capacity (A*hr, 1xN table)"; Em_LUT "Em open-circuit voltage, Em (volts, MxN table)"; R0_LUT "R0 terminal resistance (ohms, MxN table)"; R1_LUT "R1 cell resistance (ohms, MxN table)"; C1_LUT "C1 capacitance (farads, MxN table)"; cell_mass "Cell mass (kg)"; cell_Cp_heat "Cell specific heat (J/kg/K)"; SOC_LUT "SOC table breakpoints (Mx1 array)"; Temperature_LUT "Temperature table breakpoints (K, 1xN array)"
      mask DialogControl ParameterTabVar0 Prompt: Main
      mask DialogControl ParameterTabVar01 Prompt: Electrical (per cell)
      mask DialogControl ParameterTabVar012 Prompt: Thermal (per cell)
      mask DialogControl ParameterTabVar0123 Prompt: Table Breakpoints
      mask Display:
      | % Battery icon
      | plot([2.8 1.3], [0 0])
      | plot([-0.2 -1.2 -1.2 -2.8], [0 0 -0.8 -0.8])
      | patch([1 1 -1 -1]*0.15 + 1.6, [-1 1 1 -1]*0.4, [0 0 0])
      | patch([1 1 -1 -1]*0.15 + 0.4, [-1 1 1 -1]*0.4, [0 0 0])
      | patch([1 1 -1 -1]*0.15 + 1.0, [-1 1 1 -1]*0.8, [0 0 0])
      | patch([1 1 -1 -1]*0.15 - 0.2, [-1 1 1 -1]*0.8, [0 0 0])
      | 
      | % Thermal port
      | plot([-1.4 -0.8], [1.2 1.2])
      | plot([-1.4 -0.8], [0.5 0.5])
      | plot([-1.4 -2.8], [0.8 0.8])
      | plot(0.2*sin(0:2*pi/50:2*pi) - 1.4, 0.35*cos(0:2*pi/50:2*pi) + 0.85)
      | plot(0.2*sin(0:2*pi/50:pi) - 0.8, 0.35*cos(0:2*pi/50:pi) + 0.85)
      | 
      | % Plot points to set plot range
      | color('white')
      | plot(2.8, 1.6)
      | plot(-2.8, -1.6)
      | 
      | % Port labels
      | color('red')
      | port_label('LConn', 1, 'H')
      | port_label('LConn', 2, '+')
      | port_label('RConn', 1, '-')
  Pack 4 : Subsystem  mask(Lithium cell (one RC-branch equivalent circuit)){Ncells=battery_N_cells, Qe_init=battery_Qe_init, T_init=battery_T_init + 273.15, Capacity_LUT=battery_capacity_LUT, Em_LUT=battery_Em_LUT, R0_LUT=battery_R0_LUT, R1_LUT=battery_R1_LUT, C1_LUT=battery_C1_LUT, cell_mass=battery_cell_mass, cell_Cp_heat=battery_cell_cp, SOC_LUT=battery_SOC_LUT, Temperature_LUT=battery_temperature_LUT + 273.15}
      mask prompts: Ncells "Number of series-connected cells"; Qe_init "Initial cell charge deficit (A*hr)"; T_init "Initial cell temperature (K)"; Capacity_LUT "Capacity (A*hr, 1xN table)"; Em_LUT "Em open-circuit voltage, Em (volts, MxN table)"; R0_LUT "R0 terminal resistance (ohms, MxN table)"; R1_LUT "R1 cell resistance (ohms, MxN table)"; C1_LUT "C1 capacitance (farads, MxN table)"; cell_mass "Cell mass (kg)"; cell_Cp_heat "Cell specific heat (J/kg/K)"; SOC_LUT "SOC table breakpoints (Mx1 array)"; Temperature_LUT "Temperature table breakpoints (K, 1xN array)"
      mask DialogControl ParameterTabVar0 Prompt: Main
      mask DialogControl ParameterTabVar01 Prompt: Electrical (per cell)
      mask DialogControl ParameterTabVar012 Prompt: Thermal (per cell)
      mask DialogControl ParameterTabVar0123 Prompt: Table Breakpoints
      mask Display:
      | % Battery icon
      | plot([2.8 1.3], [0 0])
      | plot([-0.2 -1.2 -1.2 -2.8], [0 0 -0.8 -0.8])
      | patch([1 1 -1 -1]*0.15 + 1.6, [-1 1 1 -1]*0.4, [0 0 0])
      | patch([1 1 -1 -1]*0.15 + 0.4, [-1 1 1 -1]*0.4, [0 0 0])
      | patch([1 1 -1 -1]*0.15 + 1.0, [-1 1 1 -1]*0.8, [0 0 0])
      | patch([1 1 -1 -1]*0.15 - 0.2, [-1 1 1 -1]*0.8, [0 0 0])
      | 
      | % Thermal port
      | plot([-1.4 -0.8], [1.2 1.2])
      | plot([-1.4 -0.8], [0.5 0.5])
      | plot([-1.4 -2.8], [0.8 0.8])
      | plot(0.2*sin(0:2*pi/50:2*pi) - 1.4, 0.35*cos(0:2*pi/50:2*pi) + 0.85)
      | plot(0.2*sin(0:2*pi/50:pi) - 0.8, 0.35*cos(0:2*pi/50:pi) + 0.85)
      | 
      | % Plot points to set plot range
      | color('white')
      | plot(2.8, 1.6)
      | plot(-2.8, -1.6)
      | 
      | % Port labels
      | color('red')
      | port_label('LConn', 1, 'H')
      | port_label('LConn', 2, '+')
      | port_label('RConn', 1, '-')
  SB1 : Subsystem
  SB2 : Subsystem
  SB3 : Subsystem
  SB4 : Subsystem
  SC3 : Subsystem
  SC4 : Subsystem
  Simulink-PS Converter : nesl_utility/Simulink-PS Converter  PhysicalDomain=network_engine_domain  SubClassName=ps_input  LeftPortType=input  RightPortType=output  PseudoPeriodic=off  Frequencies=[]  NoiseDistribution=none  NoiseParameters=[]  Unit=A  AffineConversion=off  FilteringAndDerivatives=provide  SimscapeFilterOrder=1  InputFilterTimeConstant=0.001  UdotUserProvided=0
  Voltage Sensor : fl_lib/Electrical/Electrical Sensors/Voltage Sensor
  B : PMIOPort  Side=Left
  A : PMIOPort  Port=2  Side=Right
  wires:
  [I_battery] -> Simulink-PS Converter/1
  connections:
  Coolant Jacket 2/LConn1 -- Coolant Jacket 3/LConn1 -- SC3/RConn1 -- Coolant Jacket 4/LConn1 -- Coolant Jacket 1/LConn1
  Coolant Jacket 1/RConn1 -- Coolant Jacket 3/RConn1 -- SC4/LConn1 -- Coolant Jacket 4/RConn1 -- Coolant Jacket 2/RConn1
  Electrical Reference/LConn1 -- Current Demand/LConn1 -- Pack 4/RConn1 -- Voltage Sensor/RConn2
  Voltage Sensor/LConn1 -- Current Demand/RConn2 -- Pack 1/LConn2
  SC3/LConn1 -- A/RConn1
  Simulink-PS Converter/RConn1 -- Current Demand/RConn1
  SB3/LConn1 -- Pack 3/LConn1
  SB1/LConn1 -- Pack 1/LConn1
  Pack 3/LConn2 -- Pack 2/RConn1
  Pack 4/LConn2 -- Pack 3/RConn1
  SB2/RConn1 -- Coolant Jacket 2/LConn2
  Pack 1/RConn1 -- Pack 2/LConn2
  Flow Resistance (TL)/RConn1 -- B/RConn1
  SB2/LConn1 -- Pack 2/LConn1
  SB1/RConn1 -- Coolant Jacket 1/LConn2
  SB4/RConn1 -- Coolant Jacket 4/LConn2
  SB3/RConn1 -- Coolant Jacket 3/LConn2
  SB4/LConn1 -- Pack 4/LConn1
  SC4/RConn1 -- Flow Resistance (TL)/LConn1
